simulink model "control"  (R2022b)
settings: Solver=VariableStepAuto  StartTime=0.0  StopTime=200  RelTol=1e-3
libraries: slpidlib x1, simulink x1
settings Model: Creator=Aoun Raza  LastModifiedBy=Aoun Raza

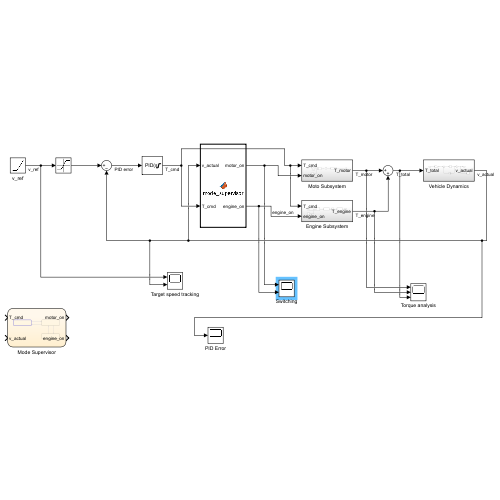
[thumbnail: Simulink's stored preview of the top-level diagram]
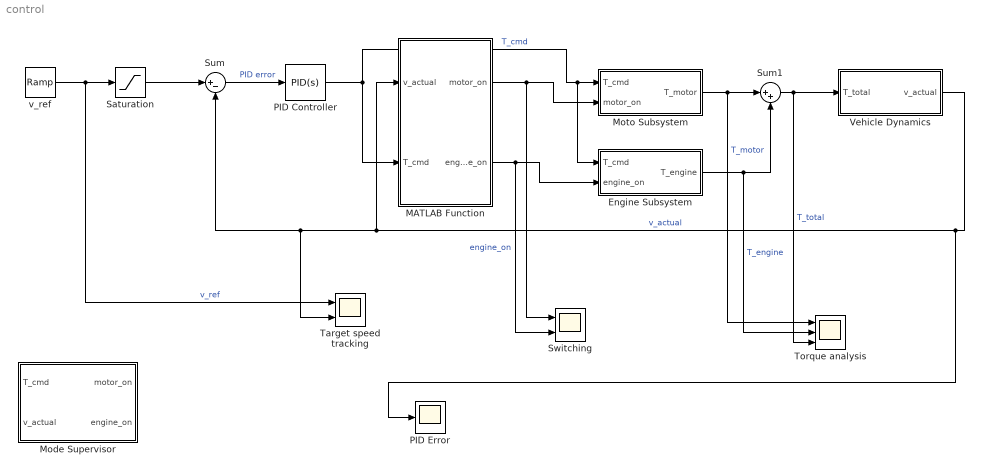
== system control ==
  Engine Subsystem : Subsystem
  MATLAB Function : MATLAB Function  TreatAsAtomicUnit=on
  Mode Supervisor : Stateflow chart  TreatAsAtomicUnit=on
  Moto Subsystem : Subsystem
  PID Controller : slpidlib/PID Controller  Controller=PID  Form=Parallel  TimeDomain=Continuous-time  UseExternalTs=off  SampleTime=-1  IntegratorMethod=Forward Euler  FilterMethod=Forward Euler  ControllerParametersSource=internal  P=528357.865419623  I=7289332.86426662  UseKiTs=off  D=7639.89930742948  N=177.313300299928  UseFilter=on  TunerSelectOption=Transfer Function Based (PID Tuner App)  InitialConditionSource=internal  InitialConditionForIntegrator=0  InitialConditionForFilter=0  DifferentiatorICPrevScaledInput=0  ExternalReset=none  TrackingMode=off  Kt=1  LimitOutput=on  SatLimitsSource=internal  UpperSaturationLimit=500  LowerSaturationLimit=0  LinearizeAsGain=on  AntiWindupMode=none  Kb=1  LimitIntegrator=off  UpperIntegratorSaturationLimit=inf  LowerIntegratorSaturationLimit=-inf  POutMin=[]  POutMax=[]  IOutMin=[]  IOutMax=[]  DOutMin=[]  DOutMax=[]  NOutMin=[]  NOutMax=[]  SumOutMin=[]  SumOutMax=[]  SaturationOutMin=[]  SaturationOutMax=[]  PParamMin=[]  PParamMax=[]  IParamMin=[]  IParamMax=[]  DParamMin=[]  DParamMax=[]  NParamMin=[]  NParamMax=[]  KbParamMin=[]  KbParamMax=[]  KtParamMin=[]  KtParamMax=[]  KbOutMin=[]  KbOutMax=[]  KtOutMin=[]  KtOutMax=[]  IntegratorOutMin=[]  IntegratorOutMax=[]  FilterOutMin=[]  FilterOutMax=[]  SumI1OutMin=[]  SumI1OutMax=[]  SumI2OutMin=[]  SumI2OutMax=[]  SumI3OutMin=[]  SumI3OutMax=[]  SumI4OutMin=[]  SumI4OutMax=[]  SumDOutMin=[]  SumDOutMax=[]  DifferentiatorOutMin=[]  DifferentiatorOutMax=[]  FilterDiffOutCoefMin=[]  FilterDiffOutCoefMax=[]  ReciprocalOutMin=[]  ReciprocalOutMax=[]  SumDenOutMin=[]  SumDenOutMax=[]  SumNumOutMin=[]  SumNumOutMax=[]  DivideOutMin=[]  DivideOutMax=[]  UdiffTsProdOutMin=[]  UdiffTsProdOutMax=[]  NTsProdOutMin=[]  NTsProdOutMax=[]  UintegralTsProdOutMin=[]  UintegralTsProdOutMax=[]  UngainTsProdOutMin=[]  UngainTsProdOutMax=[]  ClampingZeroOutDataTypeStr=Inherit: Inherit via back propagation  ClampingZeroOutMin=[]  ClampingZeroOutMax=[]  FilterDenConstantOutDataTypeStr=Inherit: Inherit via back propagation  FilterDenConstantOutMin=[]  FilterDenConstantOutMax=[]  PCopyOutDataTypeStr=Inherit: Inherit via back propagation  PCopyOutMin=[]  PCopyOutMax=[]  NCopyOutDataTypeStr=Inherit: Inherit via back propagation  NCopyOutMin=[]  NCopyOutMax=[]  IntegratorContinuousStateAttributes=''  IntegratorStateMustResolveToSignalObject=off  IntegratorRTWStateStorageClass=Auto  FilterContinuousStateAttributes=''  FilterStateMustResolveToSignalObject=off  FilterRTWStateStorageClass=Auto  ParallelPVariant=InternalParameters  IdealPVariant=Disabled  IVariant=InternalParameters  DVariant=InternalParameters  IntegratorVariant=Continuous  SatVariant=Enabled  AWVariant=Passthrough  PCopyVariant=Disabled  TRVariant=Disabled  FdbkBlocksVariant=Forward  IdealPFdbkVariant=Disabled  SatFdbkVariant=Disabled  DerivativeFilterVariant=ContFilter  NVariant=InternalParameters  NCopyVariant=Disabled  FilterICVariant=InternalICsFilter  IntegratorICVariant=InternalICs  ExternalResetVariant=Disabled  TRSumVariant=Passthrough  SumFdbkVariant=Disabled  SumVariant=Sum_PID  TsampFilterVariant=InternalTs  TsampNgainVariant=Passthrough  TsampIntegralVariant=Passthrough  ExternalSaturationOutDataTypeStr=Inherit: Same as second input
  PID Error : Scope
  Saturation : Saturate  UpperLimit=150  LowerLimit=0
  Sum : Sum  Inputs=|+-
  Sum1 : Sum  Inputs=|++
  Switching : Scope  NumInputPorts=2
  Target speed tracking : Scope  NumInputPorts=2
  Torque analysis : Scope  NumInputPorts=3
  Vehicle Dynamics : Subsystem
  v_ref : simulink/Sources/Ramp  slope=2.22  start=0  InitialOutput=0
  wires:
  Saturation/1 -> Sum/1
  PID Controller/1 -> MATLAB Function/2(T_cmd), Engine Subsystem/1(T_cmd), Moto Subsystem/1(T_cmd)  "T_cmd"
  MATLAB Function/1(motor_on) -> Switching/1, Moto Subsystem/2(motor_on)
  MATLAB Function/2(engine_on) -> Engine Subsystem/2(engine_on), Switching/2  "engine_on"
  Moto Subsystem/1(T_motor) -> Torque analysis/1, Sum1/1  "T_motor"
  Engine Subsystem/1(T_engine) -> Torque analysis/2, Sum1/2  "T_engine"
  Sum1/1 -> Torque analysis/3, Vehicle Dynamics/1(T_total)  "T_total"
  Vehicle Dynamics/1(v_actual) -> PID Error/1, Target speed tracking/2, Sum/2, MATLAB Function/1(v_actual)  "v_actual"
  v_ref/1 -> Target speed tracking/1, Saturation/1  "v_ref"
  Sum/1 -> PID Controller/1  "PID error"

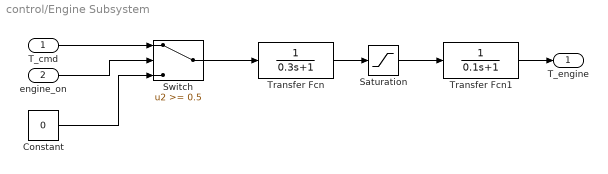
== system control/Engine Subsystem ==
  T_cmd : Inport
  engine_on : Inport  Port=2
  Constant : Constant  Value=0
  Saturation : Saturate  UpperLimit=500  LowerLimit=0
  Switch : Switch  Threshold=0.5  SaturateOnIntegerOverflow=off  InputSameDT=off
  Transfer Fcn : TransferFcn  Denominator=[0.3 1]
  Transfer Fcn1 : TransferFcn  Denominator=[0.1 1]
  T_engine : Outport
  wires:
  T_cmd/1 -> Switch/1
  engine_on/1 -> Switch/2
  Constant/1 -> Switch/3
  Switch/1 -> Transfer Fcn/1
  Transfer Fcn/1 -> Saturation/1
  Saturation/1 -> Transfer Fcn1/1
  Transfer Fcn1/1 -> T_engine/1

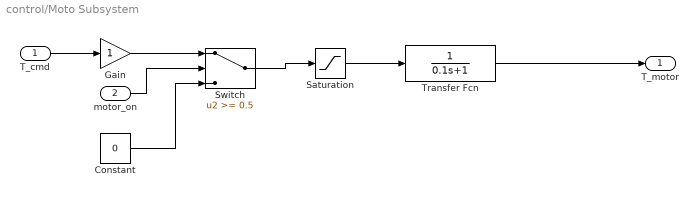
== system control/Moto Subsystem ==
  T_cmd : Inport
  motor_on : Inport  Port=2
  Constant : Constant  Value=0
  Gain : Gain
  Saturation : Saturate  UpperLimit=500  LowerLimit=0
  Switch : Switch  Threshold=0.5  SaturateOnIntegerOverflow=off  InputSameDT=off
  Transfer Fcn : TransferFcn  Denominator=[0.1 1]
  T_motor : Outport
  wires:
  T_cmd/1 -> Gain/1
  Switch/1 -> Saturation/1
  Saturation/1 -> Transfer Fcn/1
  Transfer Fcn/1 -> T_motor/1
  Gain/1 -> Switch/1
  motor_on/1 -> Switch/2
  Constant/1 -> Switch/3

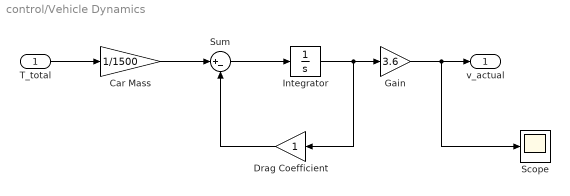
== system control/Vehicle Dynamics ==
  T_total : Inport
  Car Mass : Gain  Gain=1/1500
  Drag Coefficient : Gain
  Gain : Gain  Gain=3.6
  Integrator : Integrator
  Scope : Scope
  Sum : Sum  Inputs=|+-
  v_actual : Outport
  wires:
  T_total/1 -> Car Mass/1
  Car Mass/1 -> Sum/1
  Sum/1 -> Integrator/1
  Integrator/1 -> Drag Coefficient/1, Gain/1
  Gain/1 -> Scope/1, v_actual/1
  Drag Coefficient/1 -> Sum/2

== matlab function control/MATLAB Function ==
  data: v_actual input; motor_on output; T_cmd input; engine_on output
function [motor_on, engine_on] = mode_supervisor(v_actual, T_cmd)

if v_actual < 1000
    motor_on = 1;
    engine_on = 0;
elseif T_cmd > 200
    motor_on = 1;
    engine_on = 1;
else
    motor_on = 0;
    engine_on = 1;
end

== stateflow chart control/Mode Supervisor ==
  settings: executeAtInitialization=1
  state Engine_Mode
    entry: motor_on = 0;
    engine_on = 1;
  state EV_Mode
    entry: motor_on =1;
    engine_on = 0;
  state Boost_Mode
    entry: motor_on=1;
    engine_on = 1;
  (default) -> EV_Mode
  EV_Mode -> Engine_Mode : [v_actual>= 65]
  Engine_Mode -> EV_Mode [order 1] : [v_actual< 65]
  Boost_Mode -> Engine_Mode : [T_cmd<= 200]
  Engine_Mode -> Boost_Mode [order 2] : [T_cmd> 200]
  data: T_cmd input; motor_on output; engine_on output; v_actual input
